simulink model "hrg_wa_carrier"  (R2025a)
settings: Solver=ode4  StartTime=0.0  StopTime=.05  FixedStep=wa_full_step  RelTol=1e-3
PostLoadFcn:
  | addpath(fileparts(get_param('hrg_wa_carrier','FileName'))); wa_setup;
undefined symbols (not defined in the file or in its folder): wa_full_rhs, wa_p, wa_q0
settings Model: Creator=11725  LastModifiedBy=11725
settings DataIOCC: SaveOutput=off

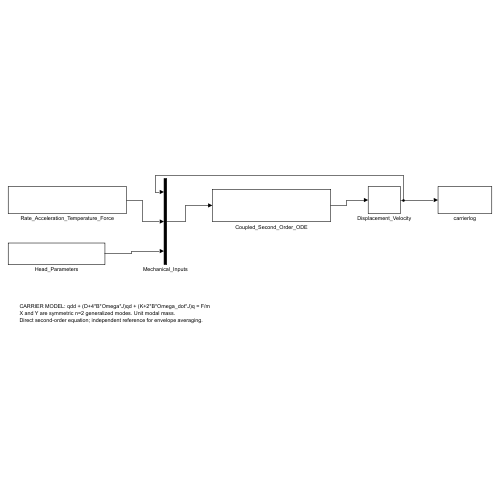
[thumbnail: Simulink's stored preview of the top-level diagram]
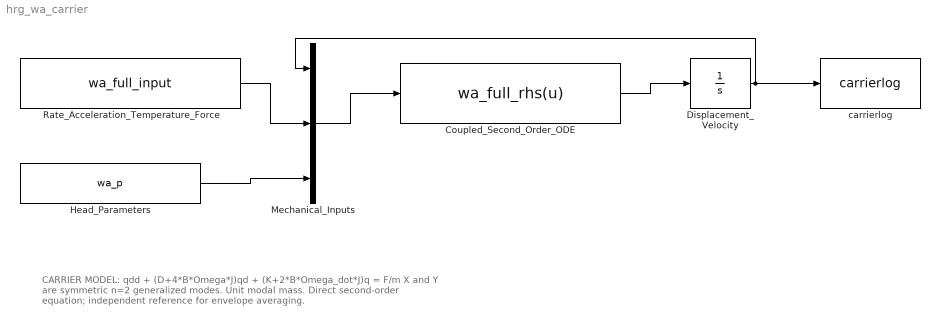
== system hrg_wa_carrier ==
  note: CARRIER MODEL: qdd + (D+4*B*Omega*J)qd + (K+2*B*Omega_dot*J)q = F/m
      | X and Y are symmetric n=2 generalized modes. Unit modal mass.
      | Direct second-order equation; independent reference for envelope averaging.
  Coupled_Second_Order_ODE : MATLABFcn  MATLABFcn=wa_full_rhs(u)  OutputDimensions=4
  Displacement_Velocity : Integrator  InitialCondition=wa_q0
  Head_Parameters : Constant  Value=wa_p
  Mechanical_Inputs : Mux  Inputs=3
  Rate_Acceleration_Temperature_Force : FromWorkspace  VariableName=wa_full_input
  carrierlog : ToWorkspace  VariableName=carrierlog  SaveFormat=Timeseries  SampleTime=-1
  wires:
  Displacement_Velocity/1 -> Mechanical_Inputs/1, carrierlog/1
  Rate_Acceleration_Temperature_Force/1 -> Mechanical_Inputs/2
  Head_Parameters/1 -> Mechanical_Inputs/3
  Mechanical_Inputs/1 -> Coupled_Second_Order_ODE/1
  Coupled_Second_Order_ODE/1 -> Displacement_Velocity/1
